simulink model "s_b4a4x1kf"  (R2018a)
settings: Solver=VariableStepDiscrete  StartTime=0.0  StopTime=1  RelTol=1e-3
undefined symbols (not defined in the file): fft_stages, n_bits_ants, n_bits_xengs
libraries: xbsIndex_r4 x22055, xbsReplacements_r4 x30, casper_library_misc x29, casper_library_scopes x15, xps_library x4
(part 70 of 227)

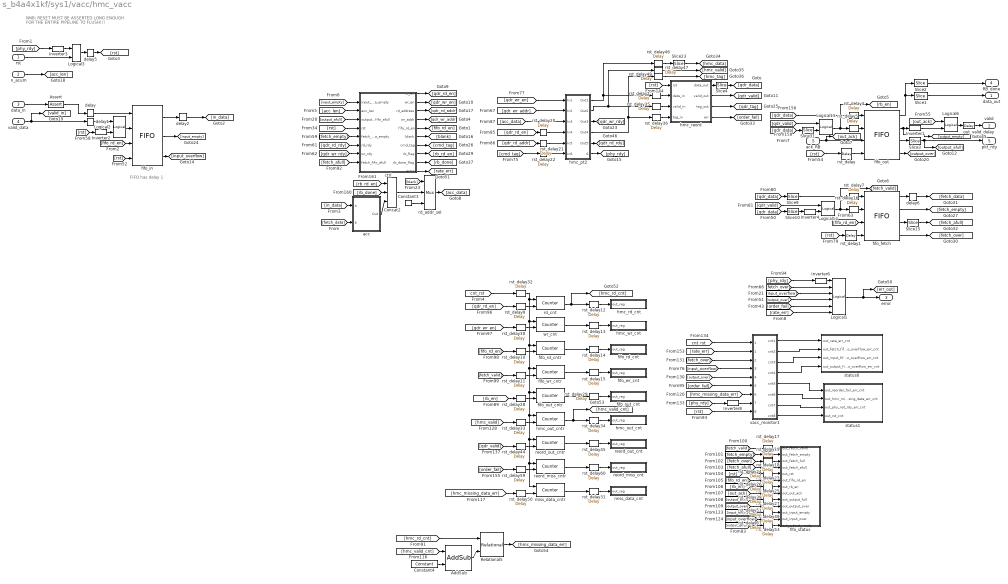
== system s_b4a4x1kf/sys1/vacc/hmc_vacc ==
  note: NNB:
      | RESET MUST BE ASSERTED LONG ENOUGH
      | FOR THE ENTIRE PIPELINE TO FLUSH!!!
  note: FIFO has delay 1
  rst : Inport
  n_acum : Inport  Port=2
  data_in : Inport  Port=3
  valid_data : Inport  Port=4
  ack_RB : Inport  Port=5
  AddSub : xbsIndex_r4/AddSub  mode=Addition  use_carryin=off  use_carryout=off  en=off  latency=1  precision=Full  arith_type=Unsigned  n_bits=16  bin_pt=14  quantization=Truncate  overflow=Wrap  use_behavioral_HDL=off  hw_selection=Fabric  pipelined=off  dbl_ovrd=off  block_type=addsub
  Assert : xbsIndex_r4/Assert  assert_type=on  type_source=Explicitly  gui_display_data_type=Fixed-point  arith_type=Unsigned  n_bits=n_bits*2^n_inputs  bin_pt=0  preci_type=Single  exp_width=8  frac_width=24  assert_rate=off  rate_source=Explicitly  period=1  output_port=on  block_type=assert
      settings: block_version=10.1.3
  Concat2 : xbsIndex_r4/Concat  num_inputs=3  dbl_ovrd=off  block_type=concat
      settings: block_version=10.1.3
  Constant3 : xbsIndex_r4/Constant  const=0  gui_display_data_type=Fixed-point  arith_type=Unsigned  n_bits=n_bits*n_inputs+2  bin_pt=0  preci_type=Single  exp_width=8  frac_width=24  explicit_period=on  period=1  equ=P=C  opselect=C  inp2=PCIN>>17  opr=+  inp1=P  carry=CIN  dbl_ovrd=off  block_type=constant
      settings: block_version=9.2.01
  Constant4 : xbsIndex_r4/Constant  const=512  gui_display_data_type=Fixed-point  arith_type=Unsigned  n_bits=10  bin_pt=0  preci_type=Single  exp_width=8  frac_width=24  explicit_period=on  period=1  equ=P=C  opselect=C  inp2=PCIN>>17  opr=+  inp1=P  carry=CIN  dbl_ovrd=off  block_type=constant
  Inverter{1..4,6} (5 alike) : xbsIndex_r4/Inverter  en=off  latency=0  dbl_ovrd=off  block_type=inv
  Inverter8 : xbsIndex_r4/Inverter  en=off  latency=2  dbl_ovrd=off  block_type=inv
  Logical1 : xbsIndex_r4/Logical  logical_function=OR  inputs=6  en=off  latency=1  precision=Full  arith_type=Unsigned  n_bits=16  bin_pt=0  align_bp=on  dbl_ovrd=off  block_type=logical
  Logical{2,6,14..15} (4 alike) : xbsIndex_r4/Logical  logical_function=AND  inputs=2  en=off  latency=0  precision=Full  arith_type=Unsigned  n_bits=16  bin_pt=0  align_bp=on  dbl_ovrd=off  block_type=logical
  Logical3 : xbsIndex_r4/Logical  logical_function=OR  inputs=2  en=off  latency=0  precision=Full  arith_type=Unsigned  n_bits=16  bin_pt=0  align_bp=on  dbl_ovrd=off  block_type=logical
  Relational5 : xbsIndex_r4/Relational  mode=a>b  op_type=Bool  en=off  latency=1  dbl_ovrd=off  block_type=relational
      settings: block_version=10.1.3
  Slice1 : xbsIndex_r4/Slice  nbits=n_bits*2^n_inputs  boolean_output=off  mode=Lower Bit Location + Width  bit1=96  base1=MSB of Input  bit0=0  base0=LSB of Input  dbl_ovrd=off  block_type=slice
      settings: block_version=9.2.01
  Slice10 : xbsIndex_r4/Slice  nbits=1  boolean_output=on  mode=Upper Bit Location + Width  bit1=0  base1=MSB of Input  bit0=-1  base0=MSB of Input  dbl_ovrd=off  block_type=slice
      settings: block_version=9.2.01
  Slice15 : xbsIndex_r4/Slice  nbits=1  boolean_output=on  mode=Upper Bit Location + Width  bit1=0  base1=MSB of Input  bit0=0  base0=LSB of Input  dbl_ovrd=off  block_type=slice
      settings: infoedit="Extracts a given range of bits from each input sample and presents it at the output.  The output type is ordinarily unsigned with binary point at zero, but can be Boolean when the slice is one bit wide.<P><P>Hardware notes: In hardware this block costs nothing."  block_version=9.2.01
  Slice2 : xbsIndex_r4/Slice  nbits=1  boolean_output=on  mode=Upper Bit Location + Width  bit1=-1  base1=MSB of Input  bit0=0  base0=LSB of Input  dbl_ovrd=off  block_type=slice
      settings: block_version=9.2.01
  Slice23 : xbsIndex_r4/Slice  nbits=(n_bits*2^n_inputs)+2  boolean_output=off  mode=Lower Bit Location + Width  bit1=96  base1=MSB of Input  bit0=0  base0=LSB of Input  dbl_ovrd=off  block_type=slice
      settings: block_version=9.2.01
  Slice3 : xbsIndex_r4/Slice  nbits=1  boolean_output=on  mode=Upper Bit Location + Width  bit1=0  base1=MSB of Input  bit0=0  base0=LSB of Input  dbl_ovrd=off  block_type=slice
      settings: infoedit="Extracts a given range of bits from each input sample and presents it at the output.  The output type is ordinarily unsigned with binary point at zero, but can be Boolean when the slice is one bit wide.<P><P>Hardware notes: In hardware this block costs nothing."  block_version=9.2.01
  Slice31 : xbsIndex_r4/Slice  nbits=1  boolean_output=on  mode=Upper Bit Location + Width  bit1=0  base1=MSB of Input  bit0=-1  base0=MSB of Input  dbl_ovrd=off  block_type=slice
      settings: block_version=9.2.01
  Slice4 : xbsIndex_r4/Slice  nbits=(n_bits*2^n_inputs)+2  boolean_output=off  mode=Lower Bit Location + Width  bit1=96  base1=MSB of Input  bit0=0  base0=LSB of Input  dbl_ovrd=off  block_type=slice
      settings: block_version=9.2.01
  Slice9 : xbsIndex_r4/Slice  nbits=(n_bits*2^n_inputs)  boolean_output=off  mode=Lower Bit Location + Width  bit1=96  base1=MSB of Input  bit0=0  base0=LSB of Input  dbl_ovrd=off  block_type=slice
      settings: block_version=9.2.01
  acc : Subsystem  mask{n_inputs=2^n_inputs, n_bits=n_bits}
      mask prompts: n_inputs "Simultaneous inputs"; n_bits "Data width"
  ctrl : Subsystem  mask{delay_fifo=2, delay_adder=2}
      mask help: QDR delay must be odd (9 is ok, 11 is ok, 10 is not).
  delay{,1..2,5..6} (5 alike) : xbsIndex_r4/Delay  rst=off  infoeditControl=Selection of Reset will increase slice count due to use of real FFs and instead of SRLs  en=off  latency=1  reg_retiming=off  dbl_ovrd=off  block_type=delay
  fifo_fetch : xbsIndex_r4/FIFO  mem_type=Block RAM  performance_options=Standard_FIFO  embedded_registers=off  depth=1K  percent_nbits=1  rst=on  rst_latency=1  en=off  use_dcount=off  use_percent_full_port=on  use_almost_empty=off  almost_empty_thresh=2  use_almost_full=off  use_rd_rst_busy=off  use_wr_rst_busy=off  almost_full_thresh=14  explicit_period=off  dbl_ovrd=off  block_type=fifo
      settings: block_version=10.1.3
  fifo_in : xbsIndex_r4/FIFO  mem_type=Block RAM  performance_options=Standard_FIFO  embedded_registers=off  depth=1K  percent_nbits=1  rst=on  rst_latency=1  en=off  use_dcount=off  use_percent_full_port=off  use_almost_empty=off  almost_empty_thresh=2  use_almost_full=off  use_rd_rst_busy=off  use_wr_rst_busy=off  almost_full_thresh=14  explicit_period=off  dbl_ovrd=off  block_type=fifo
      settings: block_version=10.1.3
  fifo_out : xbsIndex_r4/FIFO  mem_type=Block RAM  performance_options=Standard_FIFO  embedded_registers=off  depth=1K  percent_nbits=1  rst=on  rst_latency=1  en=off  use_dcount=off  use_percent_full_port=on  use_almost_empty=off  almost_empty_thresh=2  use_almost_full=off  use_rd_rst_busy=off  use_wr_rst_busy=off  almost_full_thresh=14  explicit_period=off  dbl_ovrd=off  block_type=fifo
      settings: block_version=10.1.3
  fifo_out_cnt : Subsystem  Tag=xps:sw_reg  AncestorBlock=xps_library/Memory/software_register  mask(swreg){io_dir=To Processor, io_delay=0, init_val=0, sample_period=1, names=reg, bitwidths=32, bin_pts=0, arith_types=0, sim_port=off, show_format=on}
      mask prompts: io_dir "I/O direction"; io_delay "I/O delay"; init_val "Initial Value"; sample_period "Sample period"; names "Bitfield names [msb...lsb]"; bitwidths "Bitfield widths"; bin_pts "Bitfield binary pts"; arith_types "Bitfield types, ufix=0, fix=1, bool=2"; sim_port "Provide sim input/output?"; show_format "Print format string?"
      mask help: A 32-bit software-accessible register. Can be divided into bitfields of varying widths and types using the fields in the block mask.
      mask init:
      | swreg_init(gcb)
      settings: AttributesFormatString=1output:uf32.0 = 32 bits
      mask TypeOptions io_dir: To Processor | From Processor
      mask Callback io_dir:
      | mask_enables = get_param(gcb, 'MaskEnables');
      | mask_names = get_param(gcb, 'MaskNames');
      | if strcmp(get_param(gcb, 'io_dir'), 'To Processor'),
      |     mask_enables{ismember(mask_names, 'sample_period')} = 'off';
      | else
      |     mask_enables{ismember(mask_names, 'sample_period')} = 'on';
      | end
      | set_param(gcb, 'MaskEnables', mask_enables);
      mask DialogControl ParameterTabVar0 Prompt: Setup
  fifo_out_cntr : xbsIndex_r4/Counter  cnt_type=Free Running  cnt_to=vector_len-1  operation=Up  start_count=0  cnt_by_val=1  arith_type=Unsigned  n_bits=32  bin_pt=0  load_pin=off  rst=on  en=on  explicit_period=on  period=1  use_behavioral_HDL=off  implementation=Fabric  use_rpm=off  dbl_ovrd=off  block_type=counter
  fifo_rd_cnt : Subsystem  Tag=xps:sw_reg  AncestorBlock=xps_library/Memory/software_register  mask(swreg){io_dir=To Processor, io_delay=0, init_val=0, sample_period=1, names=reg, bitwidths=32, bin_pts=0, arith_types=0, sim_port=off, show_format=on}
      mask prompts: io_dir "I/O direction"; io_delay "I/O delay"; init_val "Initial Value"; sample_period "Sample period"; names "Bitfield names [msb...lsb]"; bitwidths "Bitfield widths"; bin_pts "Bitfield binary pts"; arith_types "Bitfield types, ufix=0, fix=1, bool=2"; sim_port "Provide sim input/output?"; show_format "Print format string?"
      mask help: A 32-bit software-accessible register. Can be divided into bitfields of varying widths and types using the fields in the block mask.
      mask init:
      | swreg_init(gcb)
      settings: AttributesFormatString=1output:uf32.0 = 32 bits
      mask TypeOptions io_dir: To Processor | From Processor
      mask Callback io_dir:
      | mask_enables = get_param(gcb, 'MaskEnables');
      | mask_names = get_param(gcb, 'MaskNames');
      | if strcmp(get_param(gcb, 'io_dir'), 'To Processor'),
      |     mask_enables{ismember(mask_names, 'sample_period')} = 'off';
      | else
      |     mask_enables{ismember(mask_names, 'sample_period')} = 'on';
      | end
      | set_param(gcb, 'MaskEnables', mask_enables);
      mask DialogControl ParameterTabVar0 Prompt: Setup
  fifo_rd_cntr : xbsIndex_r4/Counter  cnt_type=Free Running  cnt_to=vector_len-1  operation=Up  start_count=0  cnt_by_val=1  arith_type=Unsigned  n_bits=32  bin_pt=0  load_pin=off  rst=on  en=on  explicit_period=on  period=1  use_behavioral_HDL=off  implementation=Fabric  use_rpm=off  dbl_ovrd=off  block_type=counter
  fifo_status : Subsystem  Tag=xps:sw_reg  AncestorBlock=xps_library/Memory/software_register  mask(swreg){io_dir=To Processor, io_delay=0, init_val=0, sample_period=1, names=[fetch_valid fetch_empty fetch_full fetch_afull rst fifo_rd_en rb_en out_ack output_full output_over input_empty input_over output_empty], bitwidths=1, bin_pts=0, arith_types=2, sim_port=off, show_format=on}
      mask prompts: io_dir "I/O direction"; io_delay "I/O delay"; init_val "Initial Value"; sample_period "Sample period"; names "Bitfield names [msb...lsb]"; bitwidths "Bitfield widths"; bin_pts "Bitfield binary pts"; arith_types "Bitfield types, ufix=0, fix=1, bool=2"; sim_port "Provide sim input/output?"; show_format "Print format string?"
      mask help: A 32-bit software-accessible register. Can be divided into bitfields of varying widths and types using the fields in the block mask.
      mask init:
      | swreg_init(gcb)
      settings: AttributesFormatString=13 outputs:b,b,b,b,b,b,b,b,b,b,b,b,b = 13 bits
      mask TypeOptions io_dir: To Processor | From Processor
      mask Callback io_dir:
      | mask_enables = get_param(gcb, 'MaskEnables');
      | mask_names = get_param(gcb, 'MaskNames');
      | if strcmp(get_param(gcb, 'io_dir'), 'To Processor'),
      |     mask_enables{ismember(mask_names, 'sample_period')} = 'off';
      | else
      |     mask_enables{ismember(mask_names, 'sample_period')} = 'on';
      | end
      | set_param(gcb, 'MaskEnables', mask_enables);
      mask DialogControl ParameterTabVar0 Prompt: Setup
  fifo_wr_cnt : Subsystem  Tag=xps:sw_reg  AncestorBlock=xps_library/Memory/software_register  mask(swreg){io_dir=To Processor, io_delay=0, init_val=0, sample_period=1, names=reg, bitwidths=32, bin_pts=0, arith_types=0, sim_port=off, show_format=on}
      mask prompts: io_dir "I/O direction"; io_delay "I/O delay"; init_val "Initial Value"; sample_period "Sample period"; names "Bitfield names [msb...lsb]"; bitwidths "Bitfield widths"; bin_pts "Bitfield binary pts"; arith_types "Bitfield types, ufix=0, fix=1, bool=2"; sim_port "Provide sim input/output?"; show_format "Print format string?"
      mask help: A 32-bit software-accessible register. Can be divided into bitfields of varying widths and types using the fields in the block mask.
      mask init:
      | swreg_init(gcb)
      settings: AttributesFormatString=1output:uf32.0 = 32 bits
      mask TypeOptions io_dir: To Processor | From Processor
      mask Callback io_dir:
      | mask_enables = get_param(gcb, 'MaskEnables');
      | mask_names = get_param(gcb, 'MaskNames');
      | if strcmp(get_param(gcb, 'io_dir'), 'To Processor'),
      |     mask_enables{ismember(mask_names, 'sample_period')} = 'off';
      | else
      |     mask_enables{ismember(mask_names, 'sample_period')} = 'on';
      | end
      | set_param(gcb, 'MaskEnables', mask_enables);
      mask DialogControl ParameterTabVar0 Prompt: Setup
  fifo_wr_cntr : xbsIndex_r4/Counter  cnt_type=Free Running  cnt_to=vector_len-1  operation=Up  start_count=0  cnt_by_val=1  arith_type=Unsigned  n_bits=32  bin_pt=0  load_pin=off  rst=on  en=on  explicit_period=on  period=1  use_behavioral_HDL=off  implementation=Fabric  use_rpm=off  dbl_ovrd=off  block_type=counter
  hmc_out_cnt : Subsystem  Tag=xps:sw_reg  AncestorBlock=xps_library/Memory/software_register  mask(swreg){io_dir=To Processor, io_delay=0, init_val=0, sample_period=1, names=reg, bitwidths=32, bin_pts=0, arith_types=0, sim_port=off, show_format=on}
      mask prompts: io_dir "I/O direction"; io_delay "I/O delay"; init_val "Initial Value"; sample_period "Sample period"; names "Bitfield names [msb...lsb]"; bitwidths "Bitfield widths"; bin_pts "Bitfield binary pts"; arith_types "Bitfield types, ufix=0, fix=1, bool=2"; sim_port "Provide sim input/output?"; show_format "Print format string?"
      mask help: A 32-bit software-accessible register. Can be divided into bitfields of varying widths and types using the fields in the block mask.
      mask init:
      | swreg_init(gcb)
      settings: AttributesFormatString=1output:uf32.0 = 32 bits
      mask TypeOptions io_dir: To Processor | From Processor
      mask Callback io_dir:
      | mask_enables = get_param(gcb, 'MaskEnables');
      | mask_names = get_param(gcb, 'MaskNames');
      | if strcmp(get_param(gcb, 'io_dir'), 'To Processor'),
      |     mask_enables{ismember(mask_names, 'sample_period')} = 'off';
      | else
      |     mask_enables{ismember(mask_names, 'sample_period')} = 'on';
      | end
      | set_param(gcb, 'MaskEnables', mask_enables);
      mask DialogControl ParameterTabVar0 Prompt: Setup
  hmc_out_cntr : xbsIndex_r4/Counter  cnt_type=Free Running  cnt_to=vector_len-1  operation=Up  start_count=0  cnt_by_val=1  arith_type=Unsigned  n_bits=32  bin_pt=0  load_pin=off  rst=on  en=on  explicit_period=on  period=1  use_behavioral_HDL=off  implementation=Fabric  use_rpm=off  dbl_ovrd=off  block_type=counter
  hmc_pt2 : Subsystem
  hmc_rd_cnt : Subsystem  Tag=xps:sw_reg  AncestorBlock=xps_library/Memory/software_register  mask(swreg){io_dir=To Processor, io_delay=0, init_val=0, sample_period=1, names=reg, bitwidths=32, bin_pts=0, arith_types=0, sim_port=off, show_format=on}
      mask prompts: io_dir "I/O direction"; io_delay "I/O delay"; init_val "Initial Value"; sample_period "Sample period"; names "Bitfield names [msb...lsb]"; bitwidths "Bitfield widths"; bin_pts "Bitfield binary pts"; arith_types "Bitfield types, ufix=0, fix=1, bool=2"; sim_port "Provide sim input/output?"; show_format "Print format string?"
      mask help: A 32-bit software-accessible register. Can be divided into bitfields of varying widths and types using the fields in the block mask.
      mask init:
      | swreg_init(gcb)
      settings: AttributesFormatString=1output:uf32.0 = 32 bits
      mask TypeOptions io_dir: To Processor | From Processor
      mask Callback io_dir:
      | mask_enables = get_param(gcb, 'MaskEnables');
      | mask_names = get_param(gcb, 'MaskNames');
      | if strcmp(get_param(gcb, 'io_dir'), 'To Processor'),
      |     mask_enables{ismember(mask_names, 'sample_period')} = 'off';
      | else
      |     mask_enables{ismember(mask_names, 'sample_period')} = 'on';
      | end
      | set_param(gcb, 'MaskEnables', mask_enables);
      mask DialogControl ParameterTabVar0 Prompt: Setup
  hmc_reord : Subsystem
  hmc_wr_cnt : Subsystem  Tag=xps:sw_reg  AncestorBlock=xps_library/Memory/software_register  mask(swreg){io_dir=To Processor, io_delay=0, init_val=0, sample_period=1, names=reg, bitwidths=32, bin_pts=0, arith_types=0, sim_port=off, show_format=on}
      mask prompts: io_dir "I/O direction"; io_delay "I/O delay"; init_val "Initial Value"; sample_period "Sample period"; names "Bitfield names [msb...lsb]"; bitwidths "Bitfield widths"; bin_pts "Bitfield binary pts"; arith_types "Bitfield types, ufix=0, fix=1, bool=2"; sim_port "Provide sim input/output?"; show_format "Print format string?"
      mask help: A 32-bit software-accessible register. Can be divided into bitfields of varying widths and types using the fields in the block mask.
      mask init:
      | swreg_init(gcb)
      settings: AttributesFormatString=1output:uf32.0 = 32 bits
      mask TypeOptions io_dir: To Processor | From Processor
      mask Callback io_dir:
      | mask_enables = get_param(gcb, 'MaskEnables');
      | mask_names = get_param(gcb, 'MaskNames');
      | if strcmp(get_param(gcb, 'io_dir'), 'To Processor'),
      |     mask_enables{ismember(mask_names, 'sample_period')} = 'off';
      | else
      |     mask_enables{ismember(mask_names, 'sample_period')} = 'on';
      | end
      | set_param(gcb, 'MaskEnables', mask_enables);
      mask DialogControl ParameterTabVar0 Prompt: Setup
  miss_data_cnt : Subsystem  Tag=xps:sw_reg  AncestorBlock=xps_library/Memory/software_register  mask(swreg){io_dir=To Processor, io_delay=0, init_val=0, sample_period=1, names=reg, bitwidths=32, bin_pts=0, arith_types=0, sim_port=off, show_format=on}
      mask prompts: io_dir "I/O direction"; io_delay "I/O delay"; init_val "Initial Value"; sample_period "Sample period"; names "Bitfield names [msb...lsb]"; bitwidths "Bitfield widths"; bin_pts "Bitfield binary pts"; arith_types "Bitfield types, ufix=0, fix=1, bool=2"; sim_port "Provide sim input/output?"; show_format "Print format string?"
      mask help: A 32-bit software-accessible register. Can be divided into bitfields of varying widths and types using the fields in the block mask.
      mask init:
      | swreg_init(gcb)
      settings: AttributesFormatString=1output:uf32.0 = 32 bits
      mask TypeOptions io_dir: To Processor | From Processor
      mask Callback io_dir:
      | mask_enables = get_param(gcb, 'MaskEnables');
      | mask_names = get_param(gcb, 'MaskNames');
      | if strcmp(get_param(gcb, 'io_dir'), 'To Processor'),
      |     mask_enables{ismember(mask_names, 'sample_period')} = 'off';
      | else
      |     mask_enables{ismember(mask_names, 'sample_period')} = 'on';
      | end
      | set_param(gcb, 'MaskEnables', mask_enables);
      mask DialogControl ParameterTabVar0 Prompt: Setup
  miss_data_cntr : xbsIndex_r4/Counter  cnt_type=Free Running  cnt_to=vector_len-1  operation=Up  start_count=0  cnt_by_val=1  arith_type=Unsigned  n_bits=32  bin_pt=0  load_pin=off  rst=on  en=on  explicit_period=on  period=1  use_behavioral_HDL=off  implementation=Fabric  use_rpm=off  dbl_ovrd=off  block_type=counter
  out_valid_delay : xbsIndex_r4/Delay  rst=off  infoeditControl=Selection of Reset will increase slice count due to use of real FFs and instead of SRLs  en=off  latency=1  reg_retiming=on  dbl_ovrd=off  block_type=delay
  rd_addr_sel : xbsIndex_r4/Mux  inputs=2  en=off  latency=0  precision=Full  arith_type=Unsigned  n_bits=16  bin_pt=14  quantization=Truncate  overflow=Wrap  dbl_ovrd=off  block_type=mux
  rd_cnt : xbsIndex_r4/Counter  cnt_type=Free Running  cnt_to=vector_len-1  operation=Up  start_count=0  cnt_by_val=1  arith_type=Unsigned  n_bits=32  bin_pt=0  load_pin=off  rst=on  en=on  explicit_period=on  period=1  use_behavioral_HDL=off  implementation=Fabric  use_rpm=off  dbl_ovrd=off  block_type=counter
  reord_miss_cnt : Subsystem  Tag=xps:sw_reg  AncestorBlock=xps_library/Memory/software_register  mask(swreg){io_dir=To Processor, io_delay=0, init_val=0, sample_period=1, names=reg, bitwidths=32, bin_pts=0, arith_types=0, sim_port=off, show_format=on}
      mask prompts: io_dir "I/O direction"; io_delay "I/O delay"; init_val "Initial Value"; sample_period "Sample period"; names "Bitfield names [msb...lsb]"; bitwidths "Bitfield widths"; bin_pts "Bitfield binary pts"; arith_types "Bitfield types, ufix=0, fix=1, bool=2"; sim_port "Provide sim input/output?"; show_format "Print format string?"
      mask help: A 32-bit software-accessible register. Can be divided into bitfields of varying widths and types using the fields in the block mask.
      mask init:
      | swreg_init(gcb)
      settings: AttributesFormatString=1output:uf32.0 = 32 bits
      mask TypeOptions io_dir: To Processor | From Processor
      mask Callback io_dir:
      | mask_enables = get_param(gcb, 'MaskEnables');
      | mask_names = get_param(gcb, 'MaskNames');
      | if strcmp(get_param(gcb, 'io_dir'), 'To Processor'),
      |     mask_enables{ismember(mask_names, 'sample_period')} = 'off';
      | else
      |     mask_enables{ismember(mask_names, 'sample_period')} = 'on';
      | end
      | set_param(gcb, 'MaskEnables', mask_enables);
      mask DialogControl ParameterTabVar0 Prompt: Setup
  reord_miss_cntr : xbsIndex_r4/Counter  cnt_type=Free Running  cnt_to=vector_len-1  operation=Up  start_count=0  cnt_by_val=1  arith_type=Unsigned  n_bits=32  bin_pt=0  load_pin=off  rst=on  en=on  explicit_period=on  period=1  use_behavioral_HDL=off  implementation=Fabric  use_rpm=off  dbl_ovrd=off  block_type=counter
  reord_out_cnt : Subsystem  Tag=xps:sw_reg  AncestorBlock=xps_library/Memory/software_register  mask(swreg){io_dir=To Processor, io_delay=0, init_val=0, sample_period=1, names=reg, bitwidths=32, bin_pts=0, arith_types=0, sim_port=off, show_format=on}
      mask prompts: io_dir "I/O direction"; io_delay "I/O delay"; init_val "Initial Value"; sample_period "Sample period"; names "Bitfield names [msb...lsb]"; bitwidths "Bitfield widths"; bin_pts "Bitfield binary pts"; arith_types "Bitfield types, ufix=0, fix=1, bool=2"; sim_port "Provide sim input/output?"; show_format "Print format string?"
      mask help: A 32-bit software-accessible register. Can be divided into bitfields of varying widths and types using the fields in the block mask.
      mask init:
      | swreg_init(gcb)
      settings: AttributesFormatString=1output:uf32.0 = 32 bits
      mask TypeOptions io_dir: To Processor | From Processor
      mask Callback io_dir:
      | mask_enables = get_param(gcb, 'MaskEnables');
      | mask_names = get_param(gcb, 'MaskNames');
      | if strcmp(get_param(gcb, 'io_dir'), 'To Processor'),
      |     mask_enables{ismember(mask_names, 'sample_period')} = 'off';
      | else
      |     mask_enables{ismember(mask_names, 'sample_period')} = 'on';
      | end
      | set_param(gcb, 'MaskEnables', mask_enables);
      mask DialogControl ParameterTabVar0 Prompt: Setup
  reord_out_cntr : xbsIndex_r4/Counter  cnt_type=Free Running  cnt_to=vector_len-1  operation=Up  start_count=0  cnt_by_val=1  arith_type=Unsigned  n_bits=32  bin_pt=0  load_pin=off  rst=on  en=on  explicit_period=on  period=1  use_behavioral_HDL=off  implementation=Fabric  use_rpm=off  dbl_ovrd=off  block_type=counter
  rst_delay{,1..2,9..15,17..19,23..36,39,44..51,53,59..60,67} (40 alike) : xbsIndex_r4/Delay  rst=off  infoeditControl=Selection of Reset will increase slice count due to use of real FFs and instead of SRLs  en=off  latency=2  reg_retiming=on  dbl_ovrd=off  block_type=delay
      rst_delay2 settings: infoedit=Hardware notes: A delay line is a chain, each link of which is an SRL16 or SRL32 followed by a flip-flop.
      rst_delay35 settings: infoedit=Hardware notes: A delay line is a chain, each link of which is an SRL16 or SRL32 followed by a flip-flop.
      rst_delay36 settings: infoedit=Hardware notes: A delay line is a chain, each link of which is an SRL16 or SRL32 followed by a flip-flop.
  rst_delay{4..5,7,16,20..22} (7 alike) : xbsIndex_r4/Delay  rst=off  infoeditControl=Selection of Reset will increase slice count due to use of real FFs and instead of SRLs  en=off  latency=1  reg_retiming=on  dbl_ovrd=off  block_type=delay
      settings: infoedit=Hardware notes: A delay line is a chain, each link of which is an SRL16 or SRL32 followed by a flip-flop.
  status0 : Subsystem  Tag=xps:sw_reg  AncestorBlock=xps_library/Memory/software_register  mask(swreg){io_dir=To Processor, io_delay=0, init_val=0, sample_period=1, names=[rate_err_cnt,fetch_fifo_overflow_err_cnt,input_fifo_overflow_err_cnt,output_fifo_overflow_err_cnt], bitwidths=8, bin_pts=0, arith_types=0, sim_port=off, show_format=on}
      mask prompts: io_dir "I/O direction"; io_delay "I/O delay"; init_val "Initial Value"; sample_period "Sample period"; names "Bitfield names [msb...lsb]"; bitwidths "Bitfield widths"; bin_pts "Bitfield binary pts"; arith_types "Bitfield types, ufix=0, fix=1, bool=2"; sim_port "Provide sim input/output?"; show_format "Print format string?"
      mask help: A 32-bit software-accessible register. Can be divided into bitfields of varying widths and types using the fields in the block mask.
      mask init:
      | swreg_init(gcb)
      settings: AttributesFormatString=4 outputs:uf8.0,uf8.0,uf8.0,uf8.0 = 32 bits
      mask TypeOptions io_dir: To Processor | From Processor
      mask Callback io_dir:
      | mask_enables = get_param(gcb, 'MaskEnables');
      | mask_names = get_param(gcb, 'MaskNames');
      | if strcmp(get_param(gcb, 'io_dir'), 'To Processor'),
      |     mask_enables{ismember(mask_names, 'sample_period')} = 'off';
      | else
      |     mask_enables{ismember(mask_names, 'sample_period')} = 'on';
      | end
      | set_param(gcb, 'MaskEnables', mask_enables);
      mask DialogControl ParameterTabVar0 Prompt: Setup
  status1 : Subsystem  Tag=xps:sw_reg  AncestorBlock=xps_library/Memory/software_register  mask(swreg){io_dir=To Processor, io_delay=0, init_val=0, sample_period=1, names=[reorder_fail_err_cnt,hmc_missing_data_err_cnt,phy_not_rdy_err_cnt,rst_cnt], bitwidths=8, bin_pts=0, arith_types=0, sim_port=off, show_format=on}
      mask prompts: io_dir "I/O direction"; io_delay "I/O delay"; init_val "Initial Value"; sample_period "Sample period"; names "Bitfield names [msb...lsb]"; bitwidths "Bitfield widths"; bin_pts "Bitfield binary pts"; arith_types "Bitfield types, ufix=0, fix=1, bool=2"; sim_port "Provide sim input/output?"; show_format "Print format string?"
      mask help: A 32-bit software-accessible register. Can be divided into bitfields of varying widths and types using the fields in the block mask.
      mask init:
      | swreg_init(gcb)
      settings: AttributesFormatString=4 outputs:uf8.0,uf8.0,uf8.0,uf8.0 = 32 bits
      mask TypeOptions io_dir: To Processor | From Processor
      mask Callback io_dir:
      | mask_enables = get_param(gcb, 'MaskEnables');
      | mask_names = get_param(gcb, 'MaskNames');
      | if strcmp(get_param(gcb, 'io_dir'), 'To Processor'),
      |     mask_enables{ismember(mask_names, 'sample_period')} = 'off';
      | else
      |     mask_enables{ismember(mask_names, 'sample_period')} = 'on';
      | end
      | set_param(gcb, 'MaskEnables', mask_enables);
      mask DialogControl ParameterTabVar0 Prompt: Setup
  vacc_monitor1 : Subsystem
  wr_cnt : xbsIndex_r4/Counter  cnt_type=Free Running  cnt_to=vector_len-1  operation=Up  start_count=0  cnt_by_val=1  arith_type=Unsigned  n_bits=32  bin_pt=0  load_pin=off  rst=on  en=on  explicit_period=on  period=1  use_behavioral_HDL=off  implementation=Fabric  use_rpm=off  dbl_ovrd=off  block_type=counter
  data_out : Outport
  valid : Outport  Port=2
  error : Outport  Port=3
  RB_done : Outport  Port=4
  pkt_rdy : Outport  Port=5
  wires:
  [rst] -> ctrl/4(rst)
  [acc_len] -> ctrl/2(acc_len)
  [output_afull] -> ctrl/3(output_fifo_afull)
  [input_empty] -> ctrl/1(input_data_empty)
  [fetch_empty] -> ctrl/5(fetch_data_empty)
  [qdr_rd_rdy] -> ctrl/6(rd_rdy)
  [qdr_wr_rdy] -> ctrl/7(wr_rdy)
  [fetch_afull] -> ctrl/8(fetch_fifo_afull)
  Logical1/1 -> [err_out], error/1
  hmc_reord/1(data_out) -> Slice4/1
  hmc_reord/2(valid_out) -> [qdr_valid]
  rst_delay2/1 -> hmc_reord/2(data_in)
  rst_delay35/1 -> hmc_reord/3(valid_in)
  rst_delay36/1 -> hmc_reord/4(tag_in)
  hmc_reord/3(tag_out) -> [qdr_tag]
  Slice4/1 -> [qdr_data]
  rst_delay46/1 -> Slice23/1
  rst_delay47/1 -> [hmc_valid]
  rst_delay48/1 -> [hmc_tag]
  [rst] -> hmc_reord/1(rst)
  hmc_reord/4(err) -> [order_fail]
  Slice23/1 -> [hmc_data]
  hmc_pt2/6(hmc_ok) -> [phy_rdy]
  [qdr_rd_en] -> rst_delay20/1
  [qdr_rd_addr] -> rst_delay21/1
  [cmd_tag] -> rst_delay22/1
  hmc_pt2/4(Out4) -> rst_delay48/1, rst_delay36/1
  hmc_pt2/1(Out1) -> rst_delay46/1, rst_delay2/1
  hmc_pt2/2(Out2) -> rst_delay47/1, rst_delay35/1
  [qdr_wr_en] -> hmc_pt2/1(In1)
  [qdr_wr_addr] -> hmc_pt2/2(In2)
  [acc_data] -> hmc_pt2/3(In3)
  rst_delay20/1 -> hmc_pt2/4(In4)
  rst_delay21/1 -> hmc_pt2/5(In5)
  rst_delay22/1 -> hmc_pt2/6(In6)
  hmc_pt2/3(Out3) -> [qdr_wr_rdy]
  hmc_pt2/5(Out5) -> [qdr_rd_rdy]
  delay5/1 -> [rst]
  n_acum/1 -> [acc_len]
  fifo_in/3 -> [input_overflow]
  fifo_in/1 -> delay2/1
  Assert/1 -> delay/1
  valid_data/1 -> delay1/1, [valid_in]
  data_in/1 -> Assert/1
  [fifo_rd_en] -> fifo_in/3
  fifo_in/2 -> [input_empty]
  delay/1 -> fifo_in/1
  Logical2/1 -> fifo_in/2
  Inverter2/1 -> Logical2/2
  [rst] -> Inverter2/1
  [rst] -> fifo_in/4
  delay2/1 -> [in_data]
  Logical3/1 -> delay5/1
  [phy_rdy] -> Inverter3/1
  rst/1 -> Logical3/2
  Inverter3/1 -> Logical3/1
  delay1/1 -> Logical2/1
  [qdr_rd_en] -> rst_delay9/1
  rd_cnt/1 -> rst_delay12/1, [hmc_rd_cnt]
  [qdr_wr_en] -> rst_delay30/1
  wr_cnt/1 -> rst_delay13/1
  [fifo_rd_en] -> rst_delay10/1
  fifo_rd_cntr/1 -> rst_delay14/1
  [fetch_valid] -> rst_delay11/1
  rst_delay12/1 -> hmc_rd_cnt/1(out_reg)
  rst_delay13/1 -> hmc_wr_cnt/1(out_reg)
  rst_delay14/1 -> fifo_rd_cnt/1(out_reg)
  rst_delay15/1 -> fifo_wr_cnt/1(out_reg)
  fifo_out_cntr/1 -> rst_delay29/1
  rst_delay29/1 -> fifo_out_cnt/1(out_reg)
  [rb_en] -> rst_delay28/1
  [cnt_rst] -> rst_delay32/1
  rst_delay32/1 -> miss_data_cntr/1, reord_miss_cntr/1, reord_out_cntr/1, hmc_out_cntr/1, fifo_out_cntr/1, fifo_wr_cntr/1, fifo_rd_cntr/1, wr_cnt/1, rd_cnt/1
  rst_delay9/1 -> rd_cnt/2
  rst_delay30/1 -> wr_cnt/2
  rst_delay10/1 -> fifo_rd_cntr/2
  rst_delay11/1 -> fifo_wr_cntr/2
  rst_delay28/1 -> fifo_out_cntr/2
  hmc_out_cntr/1 -> [hmc_valid_cnt], rst_delay34/1
  rst_delay34/1 -> hmc_out_cnt/1(out_reg)
  rst_delay33/1 -> hmc_out_cntr/2
  [hmc_valid] -> rst_delay33/1
  reord_out_cntr/1 -> rst_delay45/1
  rst_delay45/1 -> reord_out_cnt/1(out_reg)
  rst_delay44/1 -> reord_out_cntr/2
  [qdr_valid] -> rst_delay44/1
  reord_miss_cntr/1 -> rst_delay60/1
  rst_delay60/1 -> reord_miss_cnt/1(out_reg)
  rst_delay59/1 -> reord_miss_cntr/2
  [order_fail] -> rst_delay59/1
  fifo_wr_cntr/1 -> rst_delay15/1
  [hmc_rd_cnt] -> Relational5/1
  AddSub/1 -> Relational5/2
  [hmc_valid_cnt] -> AddSub/1
  Constant4/1 -> AddSub/2
  Relational5/1 -> [hmc_missing_data_err]
  [hmc_missing_data_err] -> rst_delay50/1
  rst_delay31/1 -> miss_data_cnt/1(out_reg)
  miss_data_cntr/1 -> rst_delay31/1
  rst_delay50/1 -> miss_data_cntr/2
  ctrl/6(blank) -> [blank]
  ctrl/5(fifo_rd_en) -> [fifo_rd_en]
  ctrl/3(rd_address) -> [qdr_rd_addr]
  ctrl/2(wr_en) -> [qdr_wr_en]
  ctrl/1(rd_en) -> [qdr_rd_en]
  ctrl/7(cmd_tag) -> [cmd_tag]
  ctrl/4(wr_addr) -> [qdr_wr_addr]
  ctrl/8(rb_flag) -> [rb_rd_en]
  ctrl/9(rb_done_flag) -> [rb_done]
  ctrl/10(error) -> [rate_err]
  [in_data] -> acc/1(a)
  [fetch_data] -> acc/2(b)
  fifo_out/4 -> [output_over]
  fifo_out/3 -> Slice3/1
  Slice2/1 -> RB_done/1
  fifo_out/1 -> Slice2/1, Slice1/1
  ack_RB/1 -> [out_ack], fifo_out/3
  [out_ack] -> Logical6/1
  Slice1/1 -> data_out/1
  [rst] -> rst_delay/1
  Inverter1/1 -> Logical6/2
  fifo_out/2 -> [output_empty], Inverter1/1
  Logical6/1 -> out_valid_delay/1
  rst_delay/1 -> fifo_out/4
  Slice3/1 -> pkt_rdy/1, [output_afull]
  [rst] -> rst_delay1/1
  rst_delay1/1 -> fifo_fetch/4
  [qdr_data] -> Slice9/1
  [qdr_valid] -> Logical14/1
  Slice10/1 -> Inverter4/1
  [qdr_data] -> Slice10/1
  Logical14/1 -> [fetch_valid], rst_delay16/1
  [fifo_rd_en] -> fifo_fetch/3
  Logical15/1 -> [rb_en], rst_delay5/1
  Inverter4/1 -> Logical14/2
  fifo_fetch/1 -> delay6/1
  fifo_fetch/2 -> [fetch_empty]
  fifo_fetch/4 -> [fetch_over]
  delay6/1 -> [fetch_data]
  fifo_fetch/3 -> Slice15/1
  Slice15/1 -> [fetch_afull]
  [qdr_data] -> Slice31/1
  [rb_done] -> Concat2/2
  [rb_rd_en] -> Concat2/1
  Slice9/1 -> rst_delay7/1
  acc/1(Out) -> Concat2/3
  [qdr_data] -> rst_delay4/1
  [qdr_valid] -> Logical15/1
  Slice31/1 -> Logical15/2
  rst_delay7/1 -> fifo_fetch/1
  rst_delay16/1 -> fifo_fetch/2
  Constant3/1 -> rd_addr_sel/3
  [blank] -> rd_addr_sel/1
  rd_addr_sel/1 -> [acc_data]
  Concat2/1 -> rd_addr_sel/2
  rst_delay4/1 -> fifo_out/1
  rst_delay5/1 -> fifo_out/2
  out_valid_delay/1 -> valid/1
  rst_delay23/1 -> fifo_status/4(out_fetch_afull)
  rst_delay39/1 -> fifo_status/9(out_output_full)
  [fetch_empty] -> rst_delay18/1
  [fetch_valid] -> rst_delay17/1
  [order_fail] -> vacc_monitor1/6(5)
  rst_delay53/1 -> fifo_status/12(out_input_over)
  rst_delay67/1 -> fifo_status/13(out_output_empty)
  rst_delay24/1 -> fifo_status/5(out_rst)
  vacc_monitor1/8(cnt8) -> status1/4(out_rst_cnt)
  [output_afull] -> rst_delay39/1
  rst_delay19/1 -> fifo_status/3(out_fetch_full)
  rst_delay49/1 -> fifo_status/10(out_output_over)
  [output_empty] -> rst_delay67/1
  [out_ack] -> rst_delay27/1
  rst_delay17/1 -> fifo_status/1(out_fetch_valid)
  [rst] -> vacc_monitor1/9(8)
  rst_delay25/1 -> fifo_status/6(out_fifo_rd_en)
  rst_delay18/1 -> fifo_status/2(out_fetch_empty)
  [output_over] -> vacc_monitor1/5(4)
  vacc_monitor1/5(cnt5) -> status1/1(out_reorder_fail_err_cnt)
  vacc_monitor1/3(cnt3) -> status0/3(out_input_fifo_overflow_err_cnt)
  rst_delay27/1 -> fifo_status/8(out_out_ack)
  rst_delay26/1 -> fifo_status/7(out_rb_en)
  [cnt_rst] -> vacc_monitor1/1(cnt_rst)
  [rate_err] -> vacc_monitor1/2(1)
  [rb_en] -> rst_delay26/1
  [input_overflow] -> vacc_monitor1/4(3)
  rst_delay51/1 -> fifo_status/11(out_input_empty)
  vacc_monitor1/7(cnt7) -> status1/3(out_phy_not_rdy_err_cnt)
  [fetch_over] -> rst_delay19/1
  [fetch_over] -> vacc_monitor1/3(2)
  vacc_monitor1/6(cnt6) -> status1/2(out_hmc_missing_data_err_cnt)
  [output_over] -> rst_delay49/1
  vacc_monitor1/4(cnt4) -> status0/4(out_output_fifo_overflow_err_cnt)
  [rst] -> rst_delay24/1
  [fifo_rd_en] -> rst_delay25/1
  Inverter8/1 -> vacc_monitor1/8(7)
  [hmc_missing_data_err] -> vacc_monitor1/7(6)
  [input_overflow] -> rst_delay53/1
  vacc_monitor1/2(cnt2) -> status0/2(out_fetch_fifo_overflow_err_cnt)
  [fetch_afull] -> rst_delay23/1
  [input_empty] -> rst_delay51/1
  [phy_rdy] -> Inverter8/1
  vacc_monitor1/1(cnt1) -> status0/1(out_rate_err_cnt)
  [input_overflow] -> Logical1/3
  Inverter6/1 -> Logical1/1
  [phy_rdy] -> Inverter6/1
  [order_fail] -> Logical1/5
  [output_over] -> Logical1/4
  [rate_err] -> Logical1/6
  [fetch_over] -> Logical1/2

== system s_b4a4x1kf/sys1/vacc/hmc_vacc_dummy ==
  rst : Inport
  n_acum : Inport  Port=2
  data_in : Inport  Port=3
  valid_data : Inport  Port=4
  re : Inport  Port=5
  Constant{1..4} (4 alike) : xbsIndex_r4/Constant  const=0  gui_display_data_type=Boolean  arith_type=Boolean  n_bits=248  bin_pt=0  preci_type=Single  exp_width=8  frac_width=24  explicit_period=on  period=1  equ=P=C  opselect=C  inp2=PCIN>>17  opr=+  inp1=P  carry=CIN  dbl_ovrd=off  block_type=constant
  Constant25 : xbsIndex_r4/Constant  const=0  gui_display_data_type=Fixed-point  arith_type=Unsigned  n_bits=248  bin_pt=0  preci_type=Single  exp_width=8  frac_width=24  explicit_period=on  period=1  equ=P=C  opselect=C  inp2=PCIN>>17  opr=+  inp1=P  carry=CIN  dbl_ovrd=off  block_type=constant
  data_out : Outport
  valid : Outport  Port=2
  error : Outport  Port=3
  RB_done : Outport  Port=4
  pkt_rdy : Outport  Port=5
  wires:
  Constant25/1 -> data_out/1
  Constant1/1 -> valid/1
  Constant2/1 -> error/1
  Constant3/1 -> RB_done/1
  Constant4/1 -> pkt_rdy/1

== system s_b4a4x1kf/sys1/vacc/pipeline ==
  d : Inport
  Register0 : xbsIndex_r4/Register  init=0  rst=off  en=off  dbl_ovrd=off  block_type=register
      settings: block_version=11.4
  q : Outport
  wires:
  d/1 -> Register0/1
  Register0/1 -> q/1

== system s_b4a4x1kf/sys1/vacc/status ==
  out_acc_cnt : Inport
  out_err_cnt : Inport  Port=2
  out_arm_cnt : Inport  Port=3
  out_ld_cnt : Inport  Port=4
  assert_acc_cnt : xbsIndex_r4/Assert  assert_type=on  type_source=Explicitly  gui_display_data_type=Fixed-point  arith_type=Unsigned  n_bits=12  bin_pt=0  preci_type=Single  exp_width=8  frac_width=24  assert_rate=off  rate_source=Explicitly  period=1  output_port=on  block_type=assert
  assert_arm_cnt : xbsIndex_r4/Assert  assert_type=on  type_source=Explicitly  gui_display_data_type=Fixed-point  arith_type=Unsigned  n_bits=4  bin_pt=0  preci_type=Single  exp_width=8  frac_width=24  assert_rate=off  rate_source=Explicitly  period=1  output_port=on  block_type=assert
  assert_err_cnt : xbsIndex_r4/Assert  assert_type=on  type_source=Explicitly  gui_display_data_type=Fixed-point  arith_type=Unsigned  n_bits=12  bin_pt=0  preci_type=Single  exp_width=8  frac_width=24  assert_rate=off  rate_source=Explicitly  period=1  output_port=on  block_type=assert
  assert_ld_cnt : xbsIndex_r4/Assert  assert_type=on  type_source=Explicitly  gui_display_data_type=Fixed-point  arith_type=Unsigned  n_bits=4  bin_pt=0  preci_type=Single  exp_width=8  frac_width=24  assert_rate=off  rate_source=Explicitly  period=1  output_port=on  block_type=assert
  cast_gw : xbsIndex_r4/Convert  gui_display_data_type=Fixed-point  arith_type=Unsigned  n_bits=32  bin_pt=0  float_type=Single  exp_bits=8  fraction_bits=24  quantization=Truncate  overflow=Wrap  en=off  latency=1  pipeline=off  dbl_ovrd=off  block_type=convert
  concatenate : xbsIndex_r4/Concat  num_inputs=4  dbl_ovrd=off  block_type=concat
  io_delay : xbsIndex_r4/Delay  rst=off  infoeditControl=Selection of Reset will increase slice count due to use of real FFs and instead of SRLs  en=off  latency=1  reg_retiming=on  dbl_ovrd=off  block_type=delay
  reint{1..4} (4 alike) : xbsIndex_r4/Reinterpret  force_arith_type=on  arith_type=Unsigned  force_bin_pt=on  bin_pt=0  block_type=reinterpret
  s_b4a4x1kf_sys1_vacc_status_user_data_in : xbsIndex_r4/Gateway Out  inherit_from_input=off  hdl_port=on  rows=1  columns=1  UseAsDAC=off  DACChannel='1'  interface=None  automatic_assignment=on  address_offset=hex2dec('00')  intf_name=''  intf_description=''  timing_constraint=None  locs_specified=off  LOCs={}  io_standard={}  block_type=gatewayout
  sim_out : Terminator
  wires:
  concatenate/1 -> io_delay/1
  io_delay/1 -> cast_gw/1
  cast_gw/1 -> s_b4a4x1kf_sys1_vacc_status_user_data_in/1
  s_b4a4x1kf_sys1_vacc_status_user_data_in/1 -> sim_out/1
  out_acc_cnt/1 -> assert_acc_cnt/1
  assert_acc_cnt/1 -> reint1/1
  reint1/1 -> concatenate/1
  out_err_cnt/1 -> assert_err_cnt/1
  assert_err_cnt/1 -> reint2/1
  reint2/1 -> concatenate/2
  out_arm_cnt/1 -> assert_arm_cnt/1
  assert_arm_cnt/1 -> reint3/1
  reint3/1 -> concatenate/3
  out_ld_cnt/1 -> assert_ld_cnt/1
  assert_ld_cnt/1 -> reint4/1
  reint4/1 -> concatenate/4

== system s_b4a4x1kf/sys1/vacc/timestamp ==
  out_vacc_timestamp : Inport
  assert_vacc_timestamp : xbsIndex_r4/Assert  assert_type=on  type_source=Explicitly  gui_display_data_type=Fixed-point  arith_type=Unsigned  n_bits=32  bin_pt=0  preci_type=Single  exp_width=8  frac_width=24  assert_rate=off  rate_source=Explicitly  period=1  output_port=on  block_type=assert
  cast_gw : xbsIndex_r4/Convert  gui_display_data_type=Fixed-point  arith_type=Unsigned  n_bits=32  bin_pt=0  float_type=Single  exp_bits=8  fraction_bits=24  quantization=Truncate  overflow=Wrap  en=off  latency=1  pipeline=off  dbl_ovrd=off  block_type=convert
  io_delay : xbsIndex_r4/Delay  rst=off  infoeditControl=Selection of Reset will increase slice count due to use of real FFs and instead of SRLs  en=off  latency=0  reg_retiming=on  dbl_ovrd=off  block_type=delay
  reint1 : xbsIndex_r4/Reinterpret  force_arith_type=on  arith_type=Unsigned  force_bin_pt=on  bin_pt=0  block_type=reinterpret
  s_b4a4x1kf_sys1_vacc_timestamp_user_data_in : xbsIndex_r4/Gateway Out  inherit_from_input=off  hdl_port=on  rows=1  columns=1  UseAsDAC=off  DACChannel='1'  interface=None  automatic_assignment=on  address_offset=hex2dec('00')  intf_name=''  intf_description=''  timing_constraint=None  locs_specified=off  LOCs={}  io_standard={}  block_type=gatewayout
  sim_out : Terminator
  wires:
  io_delay/1 -> cast_gw/1
  cast_gw/1 -> s_b4a4x1kf_sys1_vacc_timestamp_user_data_in/1
  s_b4a4x1kf_sys1_vacc_timestamp_user_data_in/1 -> sim_out/1
  out_vacc_timestamp/1 -> assert_vacc_timestamp/1
  assert_vacc_timestamp/1 -> reint1/1
  reint1/1 -> io_delay/1

== system s_b4a4x1kf/sys1/vacc/vacc_monitor1 ==
  cnt_rst : Inport
  new_acc : Inport  Port=2
  error : Inport  Port=3
  Delay1 : Subsystem  Tag=cmac_delinked  mask(pipeline){csp_latency=2}
      mask prompts: csp_latency "Latency"
      mask help:
      | An explicitly laid-out delay line to avoid mapping to SRL16s
      | for use in pipelining to help achieve timing closure.
      mask init:
      | pipeline_init(gcb,'latency',csp_latency);
      settings: AttributesFormatString=Latency = %<latency>
      mask Display:
      | port_label('input', 1, 'd');
      | port_label('output', 1, 'q');
      | disp(['Z^-', num2str(csp_latency)]);
  Delay121 : Subsystem  Tag=cmac_delinked  mask(pipeline){csp_latency=2}
      mask prompts: csp_latency "Latency"
      mask help:
      | An explicitly laid-out delay line to avoid mapping to SRL16s
      | for use in pipelining to help achieve timing closure.
      mask init:
      | pipeline_init(gcb,'latency',csp_latency);
      settings: AttributesFormatString=Latency = %<latency>
      mask Display:
      | port_label('input', 1, 'd');
      | port_label('output', 1, 'q');
      | disp(['Z^-', num2str(csp_latency)]);
  Delay2 : Subsystem  Tag=cmac_delinked  mask(pipeline){csp_latency=2}
      mask prompts: csp_latency "Latency"
      mask help:
      | An explicitly laid-out delay line to avoid mapping to SRL16s
      | for use in pipelining to help achieve timing closure.
      mask init:
      | pipeline_init(gcb,'latency',csp_latency);
      settings: AttributesFormatString=Latency = %<latency>
      mask Display:
      | port_label('input', 1, 'd');
      | port_label('output', 1, 'q');
      | disp(['Z^-', num2str(csp_latency)]);
  Delay25 : Subsystem  Tag=cmac_delinked  mask(pipeline){csp_latency=2}
      mask prompts: csp_latency "Latency"
      mask help:
      | An explicitly laid-out delay line to avoid mapping to SRL16s
      | for use in pipelining to help achieve timing closure.
      mask init:
      | pipeline_init(gcb,'latency',csp_latency);
      settings: AttributesFormatString=Latency = %<latency>
      mask Display:
      | port_label('input', 1, 'd');
      | port_label('output', 1, 'q');
      | disp(['Z^-', num2str(csp_latency)]);
  Delay3 : Subsystem  Tag=cmac_delinked  mask(pipeline){csp_latency=2}
      mask prompts: csp_latency "Latency"
      mask help:
      | An explicitly laid-out delay line to avoid mapping to SRL16s
      | for use in pipelining to help achieve timing closure.
      mask init:
      | pipeline_init(gcb,'latency',csp_latency);
      settings: AttributesFormatString=Latency = %<latency>
      mask Display:
      | port_label('input', 1, 'd');
      | port_label('output', 1, 'q');
      | disp(['Z^-', num2str(csp_latency)]);
  payload_cnt1 : xbsIndex_r4/Counter  cnt_type=Free Running  cnt_to=0  operation=Up  start_count=0  cnt_by_val=1  arith_type=Unsigned  n_bits=12  bin_pt=0  load_pin=off  rst=on  en=on  explicit_period=off  period=1  use_behavioral_HDL=on  implementation=Fabric  use_rpm=on  dbl_ovrd=off  block_type=counter
      settings: xl_area=[0, 0, 0, 0, 0, 0, 0]
  payload_cnt3 : xbsIndex_r4/Counter  cnt_type=Free Running  cnt_to=0  operation=Up  start_count=0  cnt_by_val=1  arith_type=Unsigned  n_bits=12  bin_pt=0  load_pin=off  rst=on  en=on  explicit_period=off  period=1  use_behavioral_HDL=on  implementation=Fabric  use_rpm=on  dbl_ovrd=off  block_type=counter
      settings: xl_area=[0, 0, 0, 0, 0, 0, 0]
  acc_cnt : Outport
  error_cnt : Outport  Port=2
  wires:
  Delay2/1(q) -> payload_cnt3/2
  payload_cnt3/1 -> Delay121/1(d)
  Delay1/1(q) -> payload_cnt1/2
  payload_cnt1/1 -> Delay25/1(d)
  cnt_rst/1 -> Delay3/1(d)
  new_acc/1 -> Delay2/1(d)
  Delay25/1(q) -> error_cnt/1
  error/1 -> Delay1/1(d)
  Delay121/1(q) -> acc_cnt/1
  Delay3/1(q) -> payload_cnt1/1, payload_cnt3/1
